simulink model "ATOM_simple_planning_simulator"  (R2026a)
settings: Solver=ode4  StopTime=100  FixedStep=0.01
StopFcn:
  | % Put every new figure in the same MATLAB Figures window as a docked tab.
  | set(groot, 'defaultFigureWindowStyle', 'docked');
  | 
  | if exist('costmap_active', 'var') && ...
  |     exist('vehicle', 'var') && ...
  |     exist('parking_path', 'var') && ...
  |     ~isempty(parking_path)
  | 
  |      plotPlan(costmap_active, vehicle, parking_path);
  | 
  |  else
  | 
  |      warning('No valid parking path is available for plotting.');
  | 
  |  end
  | 
  |  PlotControllerReferences( ...
  |      out.controller_reference_log);
  | 
  |  PlotControllerTracking( ...
  |      out.controller_tracking_log);
  | 
model workspace (MAT data in the model file):
  vehicle : object (value not decoded)
symbols that are objects in the model workspace (value not decoded): vehicle
undefined symbols (not defined in the file): delta_f_LUT, gain4WS_LUT, k_ref_LUT, kappa_gain_BP, Ki, Kp, lateral, longitudinal, planning_validator, rr_gain_BP, rr_LUT, stanley, velocity_smoother
libraries: slpidlib x1
(part 4 of 8)

== matlab function ATOM_simple_planning_simulator/trajectory_checker plugin - planning_validator_node/check_valid_steering_rate/calcMaxSteeringRates/calcSteeringAngles/steering_vector calculation ==
  data: curvature input; front_steering_vector output; rear_steering_vector output; veh input
function [front_steering_vector, rear_steering_vector] = calcSteeringVector(curvature, veh)

wheel_base = veh(3);
rear_steering_ratio = veh(29);

N = length(curvature);

front_steering_vector = zeros(N,1);
rear_steering_vector  = zeros(N,1);

for i = 1:N

    front_steering_vector(i) = ...
        CalculateFrontSteeringAngle4WS( ...
        curvature(i),...
        wheel_base,...
        rear_steering_ratio);

    rear_steering_vector(i) = rear_steering_ratio*front_steering_vector(i);
    
end
    
end

== matlab function ATOM_simple_planning_simulator/trajectory_checker plugin - planning_validator_node/HandleInvalidTrajectory - handling_type == default (case 0) ==
  data: trajectory_in input Bus: TrajectoryDataBus; trajectory_out output Bus: TrajectoryDataBus; is_valid_steering input; is_valid_steering_rate input
function trajectory_out  = ...
    HandleInvalidTrajectory( ...
    trajectory_in, ...
    is_valid_steering, ...
    is_valid_steering_rate)


% HandleInvalidTrajectory
%
% Equivalent to:
%
% PlanningValidatorNode::publishTrajectory()
%
% when:
%
% InvalidTrajectoryHandlingType::PUBLISH_AS_IT_IS
%
%
% If validation fails:
%
%   - trajectory is published unchanged
%   - validation status reports failure
%   - caution message is generated
%
%
% This reproduces Autoware behaviour.


%% ============================================================
% Validation status
% =============================================================

validation_status = ...
    is_valid_steering && is_valid_steering_rate;



%% ============================================================
% Publish trajectory behaviour
% =============================================================

% Default behaviour:
%
% PUBLISH_AS_IT_IS
%
% Therefore:
%
% output trajectory = input trajectory


trajectory_out = trajectory_in;



%% ============================================================
% Warning message
% =============================================================


if validation_status == false

     warning("Caution! Invalid Trajectory published.")

end


end

== matlab function ATOM_simple_planning_simulator/Lane Follower Scenario/Demanded trajectory generation: 90° left turn critical for 2WS --> R = 2.5 m/Trajectory Generator: 90° left turn critical for 2WS ==
  data: x output; y output; z output; qx output; qy output; qz output; qw output; longitudinal_velocity_mps output; lateral_velocity_mps output; acceleration_mps2 output; heading_rate_rps output; front_wheel_angle_rad output; rear_wheel_angle_rad output
function [x,y,z,qx,qy,qz,qw,...
          longitudinal_velocity_mps,...
          lateral_velocity_mps,...
          acceleration_mps2,...
          heading_rate_rps,...
          front_wheel_angle_rad,...
          rear_wheel_angle_rad] = trajectoryGenerator

N = 100;

%% Geometry

R = 1;              % curve radius [m]

N1 = 30;            % first straight
N2 = 40;            % circular arc
N3 = 30;            % second straight


%% Allocate outputs

x = zeros(N,1);
y = zeros(N,1);
z = zeros(N,1);

qx = zeros(N,1);
qy = zeros(N,1);
qz = zeros(N,1);
qw = zeros(N,1);

longitudinal_velocity_mps = (4/3.6)*ones(N,1);

lateral_velocity_mps = zeros(N,1);
acceleration_mps2 = zeros(N,1);
heading_rate_rps = zeros(N,1);

front_wheel_angle_rad = zeros(N,1);
rear_wheel_angle_rad = zeros(N,1);


%% ------------------------------------------------------------------------
%% First straight
%% ------------------------------------------------------------------------

L1 = 2;

for i = 1:N1

    t = (i-1)/(N1-1);

    x(i) = t*L1;
    y(i) = 0;

    yaw = 0;

    qz(i) = sin(yaw/2);
    qw(i) = cos(yaw/2);

end


%% ------------------------------------------------------------------------
%% Circular arc (90 deg)
%% ------------------------------------------------------------------------

center_x = L1;
center_y = R;

theta = linspace(-pi/2,0,N2);

for k = 1:N2

    i = N1+k;

    x(i) = center_x + R*cos(theta(k));
    y(i) = center_y + R*sin(theta(k));

    yaw = theta(k)+pi/2;

    qz(i) = sin(yaw/2);
    qw(i) = cos(yaw/2);

end


%% ------------------------------------------------------------------------
%% Second straight
%% ------------------------------------------------------------------------

L2 = 15;

x0 = x(N1+N2);
y0 = y(N1+N2);

for k = 1:N3

    i = N1+N2+k;

    t = k/(N3);

    x(i) = x0;
    y(i) = y0 + t*L2;

    yaw = pi/2;

    qz(i) = sin(yaw/2);
    qw(i) = cos(yaw/2);

end

end

== matlab function ATOM_simple_planning_simulator/Lateral run()/RearToFrontOdometry ==
  data: rear_pose input Bus: KinematicStateBus; front_pose_pred output Bus: KinematicStateBus; wheel_base input; tau_max input; d0 input; k_preview input
function front_pose_pred = RearToFrontOdometryPredictive( ...
    rear_pose,...
    wheel_base,...
    tau_max,...
    d0, k_preview)

%% ============================================================
% Predictive Rear -> Front transformation
%
% Position preview:
%   compensates steering actuator delay
%
% Orientation preview:
%   reduced anticipation for Stanley heading error
%
%% ============================================================


%% Preview times

vx = max(abs(rear_pose.twist.linear.x),0.1);

tau_pos = min(tau_max,d0/vx);

tau_yaw = k_preview*tau_pos;



%% Current rear axle state

x_r = rear_pose.pose.position.x;
y_r = rear_pose.pose.position.y;

qx = rear_pose.pose.orientation.x;
qy = rear_pose.pose.orientation.y;
qz = rear_pose.pose.orientation.z;
qw = rear_pose.pose.orientation.w;

yaw = QuaternionToYaw(qx,qy,qz,qw);



%% Vehicle velocities (body frame)

vx_body = rear_pose.twist.linear.x;
vy_body = rear_pose.twist.linear.y;

yaw_rate = rear_pose.twist.angular.z;



%% Body -> World

vx_world = ...
    vx_body*cos(yaw) - ...
    vy_body*sin(yaw);

vy_world = ...
    vx_body*sin(yaw) + ...
    vy_body*cos(yaw);



%% ============================================================
% Predict rear axle position
%% ============================================================

x_r_pred = x_r + vx_world*tau_pos;

y_r_pred = y_r + vy_world*tau_pos;



%% Orientation previews

yaw_pos  = yaw + yaw_rate*tau_pos;

yaw_ctrl = yaw + yaw_rate*tau_yaw;



%% ============================================================
% Predicted front axle position
%% ============================================================

x_f_pred = ...
    x_r_pred + wheel_base*cos(yaw_pos);

y_f_pred = ...
    y_r_pred + wheel_base*sin(yaw_pos);



%% Output

front_pose_pred = rear_pose;

front_pose_pred.pose.position.x = x_f_pred;
front_pose_pred.pose.position.y = y_f_pred;
front_pose_pred.pose.position.z = rear_pose.pose.position.z;


[qx,qy,qz,qw] = yawToQuaternion(yaw_ctrl);

front_pose_pred.pose.orientation.x = qx;
front_pose_pred.pose.orientation.y = qy;
front_pose_pred.pose.orientation.z = qz;
front_pose_pred.pose.orientation.w = qw;



%% Predicted front axle velocity (body frame)

front_pose_pred.twist.linear.x = vx_body;

front_pose_pred.twist.linear.y = ...
    vy_body + yaw_rate*wheel_base;

front_pose_pred.twist.linear.z = rear_pose.twist.linear.z;

end

== matlab function ATOM_simple_planning_simulator/Lateral run()/SetStanleyTrajectory/Resample Trajectory ==
  data: trajectory_in input Bus: TrajectoryDataBus; trajectory_out output Bus: TrajectoryDataBus; resample_interval_dist input; nearest_seg_idx input; ego_offset_to_segment input
function trajectory_out = resampleTrajectoryByDistance( ...
    trajectory_in, ...
    resample_interval_dist, ...
    nearest_seg_idx, ...
    ego_offset_to_segment)


%% ============================================================
% RESAMPLE TRAJECTORY BY ARC LENGTH
%
% Equivalent to:
%
% MPCUtils::resampleMPCTrajectoryByDistance()
%
% Adapted for Stanley controller.
%
% Unlike MPC:
% - no MPCTrajectory conversion
% - no curvature resampling
% - no optimization variables
%
% The trajectory is directly interpolated in arc length.
%
% ATTENTION:
% 
% Resampling is not actuated in Simulink since in/out buses present fixed sizes.
% See NOTE at the end of this function.
%
% =============================================================


% N = length(trajectory_in.pose.position.x);
% 
% 
% if N < 2
% 
%     trajectory_out = trajectory_in;
%     return
% 
% end
% 
% 
% 
% %% ============================================================
% % Compute arc length
% % =============================================================
% 
% x = trajectory_in.pose.position.x;
% y = trajectory_in.pose.position.y;
% 
% 
% arc_length = zeros(N,1);
% 
% 
% for i = 2:N
% 
%     dx = x(i)-x(i-1);
%     dy = y(i)-y(i-1);
% 
%     arc_length(i)= ...
%         arc_length(i-1)+sqrt(dx^2+dy^2);
% 
% end
% 
% 
% 
% if isempty(arc_length)
% 
%     trajectory_out = trajectory_in;
%     return
% 
% end
% 
% 
% 
% %% ============================================================
% % Ego position along trajectory
% %
% % Equivalent to:
% %
% % input_arclength(nearest_seg_idx)
% % + ego_offset_to_segment
% %
% % =============================================================
% 
% 
% ego_s = arc_length(nearest_seg_idx) ...
%         + ego_offset_to_segment;
% 
% 
% ego_s = min(max(ego_s,0),arc_length(end));
% 
% 
% 
% %% ============================================================
% % Generate resampling points
% %
% % Same strategy as Autoware:
% % - backward from ego
% % - forward from ego
% %
% % =============================================================
% 
% 
% output_s = [];
% 
% 
% % backward direction
% 
% s = ego_s;
% 
% while s >= 0
% 
%     output_s = [s output_s]; %#ok<AGROW>
% 
%     s = s - resample_interval_dist;
% 
% end
% 
% 
% 
% % forward direction
% 
% s = ego_s + resample_interval_dist;
% 
% 
% while s < arc_length(end)
% 
%     output_s(end+1)=s; % #ok<AGROW>
% 
%     s = s + resample_interval_dist;
% 
% end
% 
% 
% 
% %% ============================================================
% % Interpolation
% % =============================================================
% 
% 
% x_new = interp1( ...
%     arc_length,...
%     x,...
%     output_s,...
%     'linear');
% 
% 
% 
% y_new = interp1( ...
%     arc_length,...
%     y,...
%     output_s,...
%     'linear');
% 
% 
% 
% z = trajectory_in.pose.position.z;
% 
% z_new = interp1( ...
%     arc_length,...
%     z,...
%     output_s,...
%     'linear');
% 
% 
% 
% %% ============================================================
% % Quaternion / yaw interpolation
% %
% % Stanley works with yaw.
% % Therefore interpolate yaw and rebuild quaternion.
% %
% % =============================================================
% 
% 
% yaw = QuaternionToYaw( ...
%     trajectory_in.pose.orientation.qx,...
%     trajectory_in.pose.orientation.qy,...
%     trajectory_in.pose.orientation.qz,...
%     trajectory_in.pose.orientation.qw);
% 
% 
% 
% % avoid discontinuity
% 
% yaw = unwrap(yaw);
% 
% 
% 
% yaw_new = interp1( ...
%     arc_length,...
%     yaw,...
%     output_s,...
%     'linear');
% 
% 
% 
% %% ============================================================
% % Velocity interpolation
% %
% % Autoware uses linear interpolation
% % =============================================================
% 
% 
% vel_new = interp1( ...
%     arc_length,...
%     trajectory_in.longitudinal_velocity_mps,...
%     output_s,...
%     'linear');
% 
% 
% 
% lat_vel_new = interp1( ...
%     arc_length,...
%     trajectory_in.lateral_velocity_mps,...
%     output_s,...
%     'linear');
% 
% 
% 
% acc_new = interp1( ...
%     arc_length,...
%     trajectory_in.acceleration_mps2,...
%     output_s,...
%     'linear');
% 
% 
% 
% %% ============================================================
% % Build output structure
% % =============================================================
% 
% 
% M = length(output_s);
% 
% 
% trajectory_out.pose.position.x = x_new;
% trajectory_out.pose.position.y = y_new;
% trajectory_out.pose.position.z = z_new;
% 
% 
% 
% [qx,qy,qz,qw] = yawToQuaternion(yaw_new);
% 
% 
% 
% trajectory_out.pose.orientation.qx = qx;
% trajectory_out.pose.orientation.qy = qy;
% trajectory_out.pose.orientation.qz = qz;
% trajectory_out.pose.orientation.qw = qw;
% 
% 
% 
% trajectory_out.longitudinal_velocity_mps = vel_new;
% 
% trajectory_out.lateral_velocity_mps = lat_vel_new;
% 
% trajectory_out.acceleration_mps2 = acc_new;
% 
% 
% 
% % steering values are kept
% 
% trajectory_out.front_wheel_angle_rad = ...
%     interp1( ...
%     arc_length,...
%     trajectory_in.front_wheel_angle_rad,...
%     output_s,...
%     'linear');
% 
% 
% trajectory_out.rear_wheel_angle_rad = ...
%     interp1( ...
%     arc_length,...
%     trajectory_in.rear_wheel_angle_rad,...
%     output_s,...
%     'linear');
% 
% 


%% ============================================================
% NOTE (Simulink Implementation)
%
% The trajectory resampling algorithm reported above is equivalent
% to the implementation adopted by Autoware.
%
% However, the main objective of the present work is the development
% and validation of the 4WS Stanley Controller rather than the
% trajectory preprocessing module.
%
% Since Simulink requires fixed-size bus signals, the resampled
% trajectory is not generated in the simulation model.
%
% The original input trajectory is therefore directly propagated to
% the controller, preserving its fixed dimension and avoiding the
% introduction of variable-length signals.
%
% Consequently, the following assignment overwrites the resampled
% trajectory computed above.
%
% ============================================================

trajectory_out = trajectory_in;

end

== matlab function ATOM_simple_planning_simulator/Lateral run()/SetStanleyTrajectory/calcLongOffsetToSegment ==
  data: seg_idx input; ego_pose input; trajectory input Bus: TrajectoryDataBus; ego_offset_to_segment output
function ego_offset_to_segment = calcLongOffsetToSegment(seg_idx, ego_pose, trajectory)

ego_offset_to_segment = calcLongitudinalOffsetToSegment(trajectory, seg_idx, ego_pose);

end

== matlab function ATOM_simple_planning_simulator/Lateral run()/SetStanleyTrajectory/findFirstNearestSegmentIndexWithSoftConstraints ==
  data: trajectory input; dist_threshold input; yaw_threshold input; nearest_seg_idx output; pose input
function nearest_seg_idx = findNearestSegmentIndexWithSoftConstraints( ...
    trajectory, dist_threshold, yaw_threshold, pose)


%% Step 1:
% Find nearest point index

nearest_idx = findFirstNearestIndexWithSoftConstraints( ...
    trajectory, ...
    pose, ...
    dist_threshold, ...
    yaw_threshold);


N = length(trajectory.pose.position.x);


%% Step 2:
% Convert point index into segment index

% First point
if nearest_idx == 1

    nearest_seg_idx = 1;
    return

end


% Last point
if nearest_idx == N

    nearest_seg_idx = N-1;
    return

end



%% Step 3:
% Determine whether ego lies before or after nearest point
%
% Equivalent to Autoware:
%
% signed_length =
% calcLongitudinalOffsetToSegment(points,
%                                 nearest_idx,
%                                 pose.position)


signed_length = calcLongitudinalOffsetToSegment( ...
    trajectory,...
    nearest_idx,...
    pose);



%% Step 4:
% Choose segment

if signed_length <= 0

    % ego is before nearest point
    %
    % Autoware:
    % return nearest_idx - 1;

    nearest_seg_idx = nearest_idx - 1;


else

    % ego is after nearest point
    %
    % Autoware:
    % return nearest_idx;

    nearest_seg_idx = nearest_idx;

end


end

== matlab function ATOM_simple_planning_simulator/Lateral run()/MATLAB Function ==
  data: offset_limit input; enable_offset_removal input; steering_offset input; offset output
function offset = getSteeringOffset(offset_limit, enable_offset_removal, steering_offset)

persistent current_offset
if isempty(current_offset)
    current_offset = 0;
end

if enable_offset_removal
    current_offset = steering_offset;
end

offset = min(max(current_offset, -offset_limit), offset_limit);

== matlab function ATOM_simple_planning_simulator/Lateral run()/CalculateStanley/getData/calcNearestPoseInterpStanley ==
  data: self_pose input Bus: KinematicStateBus; trajectory input Bus: TrajectoryDataBus; nearest_pose output Bus: PoseBusStanley; max_dist input; max_yaw input; nearest_idx output
function [nearest_pose,nearest_idx]  = calcNearestPoseInterpStanley( ...
    self_pose, ...
    trajectory, ...
    max_dist, ...
    max_yaw)


%% ============================================================
% CALC NEAREST POSE INTERPOLATION FOR STANLEY CONTROLLER
%
% Equivalent to:
%
% MPCUtils::calcNearestPoseInterp()
%
% Differences with MPC:
%
% - Input trajectory is directly Trajectory message
% - No MPCTrajectory conversion
% - No relative_time prediction
% - Reference is already transformed to FRONT AXLE
%
% The function returns the continuous closest pose of the
% front axle on the reference trajectory.
%
% ============================================================


N = length(trajectory.pose.position.x);



%% ============================================================
% Initialization for code generation
% ============================================================

nearest_pose = struct();

nearest_pose.position.x = 0;
nearest_pose.position.y = 0;
nearest_pose.orientation.x = 0;
nearest_pose.orientation.y = 0;
nearest_pose.orientation.z = 0;
nearest_pose.orientation.w = 0;

nearest_idx = 1;

% nearest_velocity = 0;



if N == 0

    return

end



%% ============================================================
% Step 1:
% Find nearest trajectory index
%
% Equivalent to:
%
% findFirstNearestIndexWithSoftConstraints()
%
% ============================================================


nearest_idx = findFirstNearestIndexWithSoftConstraints( ...
    trajectory,...
    self_pose,...
    max_dist,...
    max_yaw);



%% ============================================================
% Single point trajectory
%
% Equivalent Autoware:
%
% if traj.size()==1
%
% ============================================================


if N == 1

    nearest_pose.x = trajectory.pose.position.x(1);
    nearest_pose.y = trajectory.pose.position.y(1);

    nearest_pose.orientation.x = trajectory.pose.orientation.qx(1);
    nearest_pose.orientation.y = trajectory.pose.orientation.qy(1);
    nearest_pose.orientation.z = trajectory.pose.orientation.qz(1);
    nearest_pose.orientation.w = trajectory.pose.orientation.qw(1);

    % nearest_velocity = trajectory.longitudinal_velocity_mps(1);

    return

end



%% ============================================================
% Step 2:
% Determine interpolation segment
%
% Equivalent to:
%
% calcLongitudinalOffset()
%
% ============================================================


if nearest_idx == 1

    prev_idx = 1;
    next_idx = 2;


elseif nearest_idx == N

    prev_idx = N-1;
    next_idx = N;


else


    p_nearest = [
        trajectory.pose.position.x(nearest_idx)
        trajectory.pose.position.y(nearest_idx)
        ];


    p_next = [
        trajectory.pose.position.x(nearest_idx+1)
        trajectory.pose.position.y(nearest_idx+1)
        ];


    signed_length = calcLongitudinalOffset( ...
        p_nearest,...
        p_next,...
        [self_pose.pose.position.x self_pose.pose.position.y]');


    if signed_length <= 0

        prev_idx = nearest_idx-1;
        next_idx = nearest_idx;

    else

        prev_idx = nearest_idx;
        next_idx = nearest_idx+1;

    end

end



%% ============================================================
% Step 3:
% Linear interpolation
%
% Equivalent to:
%
% nearest_pose.position =
% (1-ratio)*prev + ratio*next
%
% ============================================================


p_prev = [
    trajectory.pose.position.x(prev_idx)
    trajectory.pose.position.y(prev_idx)
];


p_next = [
    trajectory.pose.position.x(next_idx)
    trajectory.pose.position.y(next_idx)
];



segment_length = norm(p_next-p_prev);



% avoid division by zero

if segment_length < 1e-5


    nearest_pose.position.x = trajectory.pose.position.x(nearest_idx);
    nearest_pose.position.y = trajectory.pose.position.y(nearest_idx);


    nearest_pose.orientation.x = trajectory.pose.orientation.qx(nearest_idx);
    nearest_pose.orientation.y = trajectory.pose.orientation.qy(nearest_idx);
    nearest_pose.orientation.z = trajectory.pose.orientation.qz(nearest_idx);
    nearest_pose.orientation.w = trajectory.pose.orientation.qw(nearest_idx);

    % nearest_velocity = trajectory.longitudinal_velocity_mps(nearest_idx);


    return

end



%% Projection of ego on segment

offset = calcLongitudinalOffset( ...
    p_prev,...
    p_next,...
    [self_pose.pose.position.x self_pose.pose.position.y]');


ratio = min(max(offset / segment_length,0),1);



%% Interpolated position

nearest_pose.position.x = ...
    (1-ratio)*p_prev(1)+ratio*p_next(1);


nearest_pose.position.y = ...
    (1-ratio)*p_prev(2)+ratio*p_next(2);



%% ============================================================
% Yaw interpolation
%
% Equivalent:
%
% normalize_radian()
%
% ============================================================


yaw_prev = QuaternionToYaw( ...
    trajectory.pose.orientation.qx(prev_idx),...
    trajectory.pose.orientation.qy(prev_idx),...
    trajectory.pose.orientation.qz(prev_idx),...
    trajectory.pose.orientation.qw(prev_idx));


yaw_next = QuaternionToYaw( ...
    trajectory.pose.orientation.qx(next_idx),...
    trajectory.pose.orientation.qy(next_idx),...
    trajectory.pose.orientation.qz(next_idx),...
    trajectory.pose.orientation.qw(next_idx));


yaw_error = wrapToPi(yaw_prev-yaw_next);


nearest_yaw = wrapToPi( ...
    yaw_next + (1-ratio)*yaw_error);

[qx,qy,qz,qw] = yawToQuaternion(nearest_yaw);

nearest_pose.orientation.x = qx;
nearest_pose.orientation.y = qy;
nearest_pose.orientation.z = qz;
nearest_pose.orientation.w = qw;



% %% ============================================================
% % Velocity interpolation
% %
% % Stanley adaptation:
% %
% % The velocity is used for:
% % - gain scheduling
% % - softening factor
% %
% % ============================================================
% 
% 
% v_prev = trajectory.longitudinal_velocity_mps(prev_idx);
% 
% v_next = trajectory.longitudinal_velocity_mps(next_idx);
% 
% 
% nearest_velocity = ...
%     (1-ratio)*v_prev + ratio*v_next;


end

== matlab function ATOM_simple_planning_simulator/Lateral run()/CalculateStanley/getData/Calculate Errors/calcLateralErrorStanley ==
  data: ego_pose input Bus: KinematicStateBus; nearest_pose input Bus: PoseBusStanley; lateral_error output
function lateral_error = calcLateralErrorStanley( ...
    ego_pose, ...
    nearest_pose)


%% ============================================================
% CALC LATERAL ERROR
%
% Equivalent to Autoware:
%
% autoware::MPCUtils::calcLateralError()
%
% Computes the signed lateral distance between:
%
% - ego front axle position
% - reference front axle trajectory point
%
% Adapted for Stanley Controller.
%
% Differences with MPC:
%
% - reference trajectory is already transformed to front axle
% - no MPCTrajectory conversion
% - no additional vehicle model transformation
%
%
% Positive error:
%   vehicle is on the left side of trajectory
%
% Negative error:
%   vehicle is on the right side of trajectory
%
%
% ATTENTION!!!!!!!!!
% In Autoware, cross_track error is computed as:
% lateral_error = ...
%  -sin(ref_yaw)*err_x + ...
%      cos(ref_yaw)*err_y;
%
% by the way, in this way lat_error > 0 we the vehicle is at LHS of
% trajectory. When such error goes inside stanley controller, delta > 0 and
% the vehicle would steer more left, making the vehicle to go even further
% away from the trajectory.
%
% Therefore, lateral_error computation changes as:
%
% lateral_error = ...
    % sin(ref_yaw)*err_x - ...
    %     cos(ref_yaw)*err_y; 
%
% So that if lat_error > 0, vehicle is at RHS of the trajectory.
% ============================================================



%% Position error

err_x = ...
    ego_pose.pose.position.x - nearest_pose.position.x;


err_y = ...
    ego_pose.pose.position.y - nearest_pose.position.y;



%% Reference yaw

x = nearest_pose.orientation.x;
y = nearest_pose.orientation.y;
z = nearest_pose.orientation.z;
w = nearest_pose.orientation.w;

ref_yaw = QuaternionToYaw(x,y,z,w);



%% Projection on lateral direction

lateral_error = ...
    sin(ref_yaw)*err_x - ...
    cos(ref_yaw)*err_y;

end

== matlab function ATOM_simple_planning_simulator/Lateral run()/CalculateStanley/getData/Calculate Errors/calcYawErrorStanley ==
  data: ego_pose input Bus: KinematicStateBus; yaw_err output; nearest_pose input Bus: PoseBusStanley
function yaw_err = calcYawErrorStanley(ego_pose, nearest_pose)

%% ============================================================
% CALCULATE YAW ERROR
%
% Equivalent to:
%
% Autoware:
%
% data.yaw_err = normalize_radian(
%       tf2::getYaw(current_pose.orientation) -
%       tf2::getYaw(nearest_pose.orientation));
%
% Stanley adaptation:
%
% - current_pose refers to FRONT AXLE
% - nearest_pose is the interpolated reference pose
%   on the reference trajectory
%
% ============================================================


%% Extract yaw

qx = ego_pose.pose.orientation.x;
qy = ego_pose.pose.orientation.y;
qz = ego_pose.pose.orientation.z;
qw = ego_pose.pose.orientation.w;

x = nearest_pose.orientation.x;
y = nearest_pose.orientation.y;
z = nearest_pose.orientation.z;
w = nearest_pose.orientation.w;

current_yaw = QuaternionToYaw(qx,qy,qz,qw);

reference_yaw = QuaternionToYaw(x,y,z,w);



%% Yaw error

yaw_err = reference_yaw - current_yaw;



%% Normalize angle in [-pi, pi]

yaw_err = wrapToPi(yaw_err);


end

== matlab function ATOM_simple_planning_simulator/Parking Scenario2/Costmap generation: corridor occupancy grid/MATLAB Function ==
  data: veh input; costmap output Bus: OccupancyGridBus; start_pose output; goal_pose output
function [costmap, start_pose, goal_pose] = costmapNarrowCorridor(veh) %#ok<INUSD>
%COSTMAPNARROWCORRIDOR  8 m wide corridor.
%
% The planner turns in 5.47 m and the car is 2.66 m wide with its margin,
% so this corridor allows driving through but not turning around.
% Default task is a straight transit, which succeeds.
%
% To make it the limit case, change goal_pose heading to -pi/2 - a U-turn.
% That is expected to FAIL with a 5.47 m radius, and it is exactly the
% case a tighter turning circle would change.

persistent occ

res = 0.3;   W = 234;   H = 234;
origin_x = -(W/2)*res;
origin_y = -(H/2)*res;

if isempty(occ)
    [IX, IY] = meshgrid(0:W-1, 0:H-1);
    X = origin_x + IX*res;
    Y = origin_y + IY*res;

    lot_x = [ -4   4   4  -4];
    lot_y = [-12 -12  12  12];
    occ = ones(H,W);
    occ(inpolygon(X, Y, lot_x, lot_y)) = 0;
end

start_pose = [0, -8, pi/2];
goal_pose  = [0,  6, pi/2];

costmap.info.resolution           = res;
costmap.info.width                = uint32(W);
costmap.info.height               = uint32(H);
costmap.info.origin.position.x    = origin_x;
costmap.info.origin.position.y    = origin_y;
costmap.info.origin.position.z    = 0;
costmap.info.origin.orientation.x = 0;
costmap.info.origin.orientation.y = 0;
costmap.info.origin.orientation.z = 0;
costmap.info.origin.orientation.w = 1;
costmap.data                      = int8(occ*100);
end

== matlab function ATOM_simple_planning_simulator/Lateral run()/CalculateStanley/Stanley controller/calculateSteer - Stanley ==
  data: stanley_data input Bus: StanleyInputDataBus; wheelbase input; steer_limit input; front_steer output; k_gain input; k_soft input; rr input; gain_4WS input; rear_steer output
function [front_steer, rear_steer] = calculateSteer( ...
    stanley_data,...
    wheelbase, ...
    steer_limit, ...
    k_gain,...
    k_soft,...
    rr, ...
    gain_4WS)


%% ============================================================
% STANLEY CONTROLLER
%
% Equivalent to the lateral control law used in:
%
% Stanley 4WS:
%
% delta = (yaw_error + atan(k*e_y/(v+k_soft))) * gain_4WS
%
%
% Adaptation for Autoware:
%
% - input data are generated in getDataStanley()
% - reference trajectory is expressed at FRONT AXLE
% - current pose is expressed at FRONT AXLE
% - only front steering command is generated
%
% ============================================================


%% ============================================================
% Extract Stanley data
% ============================================================


lateral_error = stanley_data.lateral_err;

yaw_error = stanley_data.yaw_err;

vel_x = stanley_data.vel_x;

curvature = stanley_data.ref_curvature;



%% ============================================================
% Stanley lateral correction
%
% Equivalent to:
%
% atan(k*e_y/v)
%
% with softening term:
%
% atan(k*e_y/(v+k_soft))
%
% ============================================================


cross_track_term = atan2( ...
    k_gain*(lateral_error),...
    vel_x + k_soft);

%% ============================================================
% Steering command
%
% Heading correction + lateral correction
% ============================================================
yaw_error = 0;

%front_steer = (yaw_error + cross_track_term) + gain_4WS*asin(curvature*wheelbase);

front_steer = 15*cross_track_term;

%% ===========================================================
% Saturate front steer
%
% ============================================================

front_steer = min( ...
    max(front_steer,-steer_limit),...
    steer_limit);

front_steer = gain_4WS * front_steer;

%% ===========================================================
% Compute rear steer command
%
% ============================================================

rear_steer = rr * front_steer;

end

== matlab function ATOM_simple_planning_simulator/Lateral run()/CalculateStanley/Saturate steering_cmd ==
  data: steering_cmd input; steering_cmd_sat output; steer_limit input
function steering_cmd_sat = clamp(steering_cmd, steer_limit)

%% ============================================================
% Steering saturation
%
% Equivalent to MPC:
%
% std::clamp(Uex(0), -m_steer_lim, m_steer_lim)
%
% ============================================================


steering_cmd_sat = min( ...
    max(steering_cmd,-steer_limit),...
    steer_limit);



end

== matlab function ATOM_simple_planning_simulator/Lateral run()/CalculateStanley/Filter steering_cmd ==
  data: steering_cmd_sat input; steering_cmd output
function steering_cmd = filterSteerCmd(steering_cmd_sat)

% NOTE (Simulink Implementation)
% 
% In Autoware, the steering command is subsequently filtered using a 
% second-order Butterworth filter (Butterworth2dFilter) to attenuate 
% % high-frequency oscillations and produce a smoother steering input:
% 
%  const double u_filtered = m_lpf_steering_cmd.filter(u_saturated);
% 
% Since this operation is a post-processing stage independent of the adopted 
% lateral control law, it has not been implemented in the Simulink model. 
% This allows the simulation to evaluate exclusively the behavior of the 
% Stanley controller without introducing additional filtering effects.

steering_cmd = steering_cmd_sat;

== matlab function ATOM_simple_planning_simulator/Lateral run()/CalculateStanley/getData/Calculate Errors/Plot Stanley Errors ==
  settings: updateMethod=DISCRETE
  data: lateral_error input; heading_error input double
function plotErrors(lateral_error, heading_error)

persistent hFig
persistent ax
persistent hLat
persistent hHead

persistent lat_history
persistent head_history
persistent time_history

persistent k

%% ============================================================
% Initialization
%% ============================================================

if isempty(k)

    k = 1;

    lat_history = lateral_error;
    head_history = heading_error;
    time_history = 0;

    hFig = figure(10);
    clf

    ax = axes(hFig);

    hold(ax,'on')
    grid(ax,'on')

    xlabel(ax,'Sample')
    ylabel(ax,'Error')

    title(ax,'Stanley Tracking Errors')

    hLat = plot(time_history,...
        lat_history,...
        'b','LineWidth',2);

    hHead = plot(time_history,...
        head_history,...
        'r','LineWidth',2);

    legend(ax,...
        {'Lateral Error','Heading Error'},...
        'Location','best');

else

    k = k + 1;

    time_history(end+1) = k;
    lat_history(end+1) = lateral_error;
    head_history(end+1) = heading_error;

    set(hLat,...
        'XData',time_history,...
        'YData',lat_history);

    set(hHead,...
        'XData',time_history,...
        'YData',head_history);

end

xlim(ax,[0 max(100,k)])

drawnow limitrate

end

== matlab function ATOM_simple_planning_simulator/Lane Follower Scenario/Straight trajectory/Trajectory Generator: straight ==
  data: x output; y output; z output; qx output; qy output; qz output; qw output; longitudinal_velocity_mps output; lateral_velocity_mps output; acceleration_mps2 output; heading_rate_rps output; front_wheel_angle_rad output; rear_wheel_angle_rad output
function [x,y,z,qx,qy,qz,qw,...
          longitudinal_velocity_mps,...
          lateral_velocity_mps,...
          acceleration_mps2,...
          heading_rate_rps,...
          front_wheel_angle_rad,...
          rear_wheel_angle_rad] = trajectoryGenerator

N = 100;

%% Geometry


N1 = N;            % first straight



%% Allocate outputs

x = zeros(N,1);
y = zeros(N,1);
z = zeros(N,1);

qx = zeros(N,1);
qy = zeros(N,1);
qz = zeros(N,1);
qw = zeros(N,1);

longitudinal_velocity_mps = (4/3.6)*ones(N,1);

lateral_velocity_mps = zeros(N,1);
acceleration_mps2 = zeros(N,1);
heading_rate_rps = zeros(N,1);

front_wheel_angle_rad = zeros(N,1);
rear_wheel_angle_rad = zeros(N,1);


%% ------------------------------------------------------------------------
%% First straight
%% ------------------------------------------------------------------------

L1 = 50;

for i = 1:N1

    t = (i-1)/(N1-1);

    x(i) = t*L1;
    y(i) = 0;

    yaw = 0;

    qz(i) = sin(yaw/2);
    qw(i) = cos(yaw/2);

end



end

== matlab function ATOM_simple_planning_simulator/Lateral run()/CalculateStanley/Plot steer command ==
  settings: updateMethod=DISCRETE
  data: front_steer input; rear_steer input
function plotSteerCmd(front_steer, rear_steer)

persistent hFig
persistent ax
persistent hSteerFront
persistent hSteerRear

persistent steerFront_history
persistent steerRear_history
persistent time_history

persistent k

%% ============================================================
% Initialization
%% ============================================================

if isempty(k)

    k = 1;

    steerFront_history = front_steer;
    steerRear_history = rear_steer;
    time_history = 0;

    hFig = figure(11);
    clf

    ax = axes(hFig);

    hold(ax,'on')
    grid(ax,'on')

    xlabel(ax,'Sample')
    ylabel(ax,'Steering command')

    title(ax,'Steering commands')

    hSteerFront = plot(time_history,...
        steerFront_history,...
        'r','LineWidth',2);

    hSteerRear = plot(time_history,...
        steerRear_history,...
        'b','LineWidth',2);

    legend(ax,...
        {'Front steer command','Rear Steer command'},...
        'Location','best');

else

    k = k + 1;

    time_history(end+1) = k;
    steerFront_history(end+1) = front_steer;
    steerRear_history(end+1) = rear_steer;

    set(hSteerFront,...
        'XData',time_history,...
        'YData',steerFront_history);

    set(hSteerRear,...
        'XData',time_history,...
        'YData',steerRear_history);

end

xlim(ax,[0 max(100,k)])

drawnow limitrate

end

== matlab function ATOM_simple_planning_simulator/LongitudinalRun()/RearToFrontOdometry ==
  data: rear_pose input Bus: KinematicStateBus; front_pose_pred output Bus: KinematicStateBus; wheel_base input
function front_pose_pred = RearToFrontOdometryCurrent( ...
    rear_pose, ...
    wheel_base)

front_pose_pred = rear_pose;

% 1. Estrazione dello Yaw dall'orientamento (Quaternion -> Yaw)
qx = rear_pose.pose.orientation.x;
qy = rear_pose.pose.orientation.y;
qz = rear_pose.pose.orientation.z;
qw = rear_pose.pose.orientation.w;
yaw = QuaternionToYaw(qx, qy, qz, qw);

% 2. Calcolo della Posizione Attuale dell'Asse Anteriore (Mappa/World Frame)
x_front_now = rear_pose.pose.position.x + wheel_base * cos(yaw);
y_front_now = rear_pose.pose.position.y + wheel_base * sin(yaw);

% 3. Velocità dell'Asse Anteriore espresso nel Frame Veicolo (Body Frame)
v_x_body = rear_pose.twist.linear.x;
v_y_body = rear_pose.twist.linear.y + rear_pose.twist.angular.z * wheel_base;

% 4. Conversione delle Velocità dal Frame Veicolo (Body) al Frame Mappa (World)
% Ruotiamo il vettore velocità [v_x_body, v_y_body] dell'angolo yaw attuale:
v_x_world = v_x_body * cos(yaw) - v_y_body * sin(yaw);
v_y_world = v_x_body * sin(yaw) + v_y_body * cos(yaw);

% 5. PREDIZIONE TEMPORALE (Coordinate t + tau nel Frame Mappa)
front_pose_pred.pose.position.x = x_front_now;
front_pose_pred.pose.position.y = y_front_now;
front_pose_pred.pose.position.z = rear_pose.pose.position.z;

% 6. Aggiornamento delle velocità nel messaggio di output (Frame Veicolo)
front_pose_pred.twist.linear.x = v_x_body;
front_pose_pred.twist.linear.y = v_y_body;
front_pose_pred.twist.linear.z = rear_pose.twist.linear.z;

% 7. L'orientamento rimane lo stesso (o aggiornato con il pitch/roll se presente)
front_pose_pred.pose.orientation = rear_pose.pose.orientation;

end

== matlab function ATOM_simple_planning_simulator/Plot front//rear steer status ==
  settings: updateMethod=DISCRETE
  data: front_steer input; rear_steer input
function plotSteerCmd(front_steer, rear_steer)

persistent hFig
persistent ax
persistent hSteerFront
persistent hSteerRear

persistent steer_front_history
persistent steer_rear_history
persistent time_history

persistent k

%% ============================================================
% Initialization
%% ============================================================

if isempty(k)

    k = 1;

    steer_front_history = front_steer;
    steer_rear_history = rear_steer;
    time_history = 0;

    hFig = figure(12);
    clf

    ax = axes(hFig);

    hold(ax,'on')
    grid(ax,'on')

    xlabel(ax,'Sample')
    ylabel(ax,'Steering command')

    title(ax,'Front steering command')

    hSteerFront = plot(time_history,...
        steer_front_history,...
        'r','LineWidth',2);

    hSteerRear = plot(time_history, ...
        steer_rear_history, 'b', 'LineWidth', 2);

    title('Front and rear steering status')
    
    legend(ax,...
        {'Front steer status','Rear Steer Status'},...
        'Location','best');

else

    k = k + 1;

    time_history(end+1) = k;
    steer_front_history(end+1) = front_steer;
    steer_rear_history(end+1) = rear_steer;

    set(hSteerFront,...
        'XData',time_history,...
        'YData',steer_front_history);

    set(hSteerRear,...
        'XData',time_history,...
        'YData',steer_rear_history);

end

xlim(ax,[0 max(100,k)])

drawnow limitrate

end

== matlab function ATOM_simple_planning_simulator/Plot vehicle/RearToFrontOdometry ==
  data: rear_pose input Bus: KinematicStateBus; front_pose output Bus: KinematicStateBus; wheel_base input
function front_pose = RearToFrontOdometry( ...
    rear_pose,...
    wheel_base)


front_pose = rear_pose;


qx = rear_pose.pose.orientation.x;
qy = rear_pose.pose.orientation.y;
qz = rear_pose.pose.orientation.z;
qw = rear_pose.pose.orientation.w;


yaw = QuaternionToYaw(qx,qy,qz,qw);



front_pose.pose.position.x = ...
    rear_pose.pose.position.x + ...
    wheel_base*cos(yaw);


front_pose.pose.position.y = ...
    rear_pose.pose.position.y + ...
    wheel_base*sin(yaw);


front_pose.pose.position.z = ...
    rear_pose.pose.position.z;



% orientation unchanged

front_pose.pose.orientation = ...
    rear_pose.pose.orientation;


% Linear velocity referred to front axle

front_pose.twist.linear.x = rear_pose.twist.linear.x ...
    - rear_pose.twist.angular.z ...
    * wheel_base*sin(yaw);


front_pose.twist.linear.y = rear_pose.twist.linear.y ...
    + rear_pose.twist.angular.z ...
    * wheel_base*cos(yaw);


front_pose.twist.linear.z = rear_pose.twist.linear.z;


end

== matlab function ATOM_simple_planning_simulator/Lateral run()/CalculateStanley/getData/Plot Nearest Pose ==
  settings: updateMethod=DISCRETE
  data: nearest_pose input
function plotNearestPose(nearest_pose)

persistent hFig
persistent ax
persistent hX
persistent hY

persistent X_history
persistent Y_history
persistent time_history

persistent k

%% ============================================================
% Initialization
%% ============================================================

if isempty(k)

    k = 1;

    X_history = nearest_pose.position.x;
    Y_history = nearest_pose.position.x;
    time_history = 0;

    hFig = figure(14);
    clf

    ax = axes(hFig);

    hold(ax,'on')
    grid(ax,'on')

    xlabel(ax,'Sample')
    ylabel(ax,'Error')

    title(ax,'Nearest_pose')

    hX = plot(time_history,...
        X_history,...
        'b','LineWidth',2);

    hY = plot(time_history,...
        Y_history,...
        'r','LineWidth',2);

    legend(ax,...
        {'X nearest','Y nearest'},...
        'Location','best');

else

    k = k + 1;

    time_history(end+1) = k;
    X_history(end+1) = nearest_pose.position.x;
    Y_history(end+1) = nearest_pose.position.y;

    set(hX,...
        'XData',time_history,...
        'YData',X_history);

    set(hY,...
        'XData',time_history,...
        'YData',Y_history);

end

xlim(ax,[0 max(100,k)])

drawnow limitrate

end

== matlab function ATOM_simple_planning_simulator/Vehicle Model/Vehicle Dynamics/MATLAB Function ==
  data: state input Bus: VehicleInternalStateBus size=1; d_state output Bus: VehicleInternalStateBus size=1; command input Bus: ControlCMDBus size=1; veh input; rear_steering_command input
function d_state = vehicleDynamics(state, command, veh, rear_steering_command)

%%%%%%%%%%%%%%%%%%%%%%%%%%%%%%%%%%%%%%
%%%%%%%%%%%%%%%%%%%%%%%%%%%%%%%%%%%%%%
% Description:
% This vehicleDynamics model follows DELAY_STEER_ACC_GEARED
% model, it doesn't presents a model for gear management
% since its not something we're going to modify on Autoware for 4WS
% implementation.
%
% Inputs:
% - state: VehicleInternalStateBus. It contains the state of the vehicle
%          at time instant t. 
% - command: /control/command/control_cmd topic --> ControlCMDBus.
%          It contains the desired acc and steering commands coming from
%          the control region.
%
% - Parameters
% - vehicle: vehicle parameters struct defined in vehicleParameters.m.

% Outputs: 
% - d_state: It contains the derivative of the state of the vehicle at time
%          instant t+1.
%%%%%%%%%%%%%%%%%%%%%%%%%%%%%%%%%%%%%%
%%%%%%%%%%%%%%%%%%%%%%%%%%%%%%%%%%%%%%


% inside MATLAB Function: input is veh_in (1xN double)
v = veh; % 1xN numeric row

vehicle.param.wheel_radius    = v(1);
vehicle.param.wheel_width     = v(2);
vehicle.param.wheel_base      = v(3);
vehicle.param.wheel_tread     = v(4);
vehicle.param.front_overhang  = v(5);
vehicle.param.rear_overhang   = v(6);
vehicle.param.left_overhang   = v(7);
vehicle.param.right_overhang  = v(8);
vehicle.param.vehicle_height  = v(9);
vehicle.param.max_steer_angle = v(10);

% decode integer-coded enums (example)
vehicle.sim.vehicle_model_type = int32(v(11));    % or map to strings if needed
vehicle.sim.initialize_source  = int32(v(12));

vehicle.sim.timer_sampling_time_ms = v(13);
vehicle.sim.add_measurement_noise = logical(v(14));
vehicle.sim.vel_lim        = v(15);
vehicle.sim.vel_rate_lim   = v(16);
vehicle.sim.steer_lim      = v(17);
vehicle.sim.steer_rate_lim = v(18);
vehicle.sim.acc_time_delay = v(19);
vehicle.sim.acc_time_constant = v(20);
vehicle.sim.steer_time_delay   = v(21);
vehicle.sim.steer_time_constant= v(22);
vehicle.sim.x_stddev = v(23);
vehicle.sim.y_stddev = v(24);
vehicle.sim.steer_dead_band = v(25);
vehicle.sim.steer_bias = v(26);
vehicle.sim.debug_acc_scaling_factor = v(27);
vehicle.sim.debug_steer_scaling_factor = v(28);

% Parameter for 4WS
vehicle.param.rear_steering_ratio = veh(29);
rear_steering_ratio = vehicle.param.rear_steering_ratio;

%% ==========================
% Saturation function
% ===========================

sat = @(val, upper, lower) min(max(val,lower),upper);



%% ==========================
% Current state
% ===========================

vx = sat( ...
    state.vx,...
    vehicle.sim.vel_lim,...
   -vehicle.sim.vel_lim);


acc = sat( ...
    state.acc,...
    vehicle.sim.vel_rate_lim,...
   -vehicle.sim.vel_rate_lim);


yaw = state.yaw;

steer_front = state.steer_front;
steer_rear = state.steer_rear;          % Modified for 4WS  


%% ==========================
% Input commands
% ===========================

acc_des = sat( ...
    command.longitudinal.acceleration,...
    vehicle.sim.vel_rate_lim,...
   -vehicle.sim.vel_rate_lim);


acc_des = acc_des * ...
    vehicle.sim.debug_acc_scaling_factor;



steer_front_des = sat( ...
    command.lateral.steering_tire_angle,...
    vehicle.sim.steer_lim,...
   -vehicle.sim.steer_lim);


steer_front_des = steer_front_des * ...
    vehicle.sim.debug_steer_scaling_factor;

steer_rear_des = sat( ...                                            % Modified for 4WS
    rear_steering_command,...
    vehicle.sim.steer_lim,...
    -vehicle.sim.steer_lim);


steer_rear_des = steer_rear_des * ...                                % Modified for 4WS
    vehicle.sim.debug_steer_scaling_factor;



%% ==========================
% Steering dynamics
% ===========================

% getSteer() in simple_planning_simulator corresponds to state.steer
% From the phisical vehicle front_steer and rear_steer are measured.

steer_diff_front = steer_front - steer_front_des;

steer_diff_rear = steer_rear  - steer_rear_des;             % Modified for 4WS


% dead band

if steer_diff_front > vehicle.sim.steer_dead_band

    steer_diff_with_dead_band_front = ...
        steer_diff_front - vehicle.sim.steer_dead_band;


elseif steer_diff_front < -vehicle.sim.steer_dead_band

    steer_diff_with_dead_band_front = ...
        steer_diff_front + vehicle.sim.steer_dead_band;


else

    steer_diff_with_dead_band_front = 0;

end



if steer_diff_rear > vehicle.sim.steer_dead_band            % Modified for 4WS

    steer_diff_with_dead_band_rear = ...
        steer_diff_rear - vehicle.sim.steer_dead_band;


elseif steer_diff_rear < -vehicle.sim.steer_dead_band

    steer_diff_with_dead_band_rear = ...
        steer_diff_rear + vehicle.sim.steer_dead_band;


else

    steer_diff_with_dead_band_rear = 0;

end



steer_rate_front = sat( ...
    -steer_diff_with_dead_band_front / vehicle.sim.steer_time_constant,...
     vehicle.sim.steer_rate_lim,...
    -vehicle.sim.steer_rate_lim);

steer_rate_rear = sat( ...                                                  % Modified for 4WS
    -steer_diff_with_dead_band_rear / vehicle.sim.steer_time_constant,...
    vehicle.sim.steer_rate_lim,...
    -vehicle.sim.steer_rate_lim);



%% ==========================
% State derivative
% ===========================

%--------------------------------------------------------------
% 4WS kinematic bicycle model
%
% Assumptions:
%   - Pure rolling
%   - alpha_f = alpha_r = 0
%   - No tire dynamics
%   - No lateral slip dynamics
%
% beta is the geometric vehicle sideslip angle. Since Autoware defines
% reference frame of the vehicle equal to centre of the rear axle, then
% beta = steer_rear
%--------------------------------------------------------------

L = vehicle.param.wheel_base;


beta = steer_rear;                              % Modified for 4WS


vel = vx/cos(beta);                             % Modified for 4WS


yaw_rate = ...                                  % Modified for 4WS
    (vx/L) * ...
    (tan(steer_front)-tan(steer_rear));


d_state.x = vel*cos(yaw + beta);                % Modified for 4WS

d_state.y = vel*sin(yaw + beta);                % Modified for 4WS


d_state.yaw = yaw_rate;                         % Modified for 4WS


d_state.vx = acc + yaw_rate*vel*sin(beta);


d_state.steer_front = steer_rate_front;

d_state.steer_rear = steer_rate_rear;           % Modified for 4WS

d_state.acc = ...
    -(acc-acc_des)/vehicle.sim.acc_time_constant;

end
